simulink model "buck_ls_fault_sw_4rt"  (R2025a)
settings: Solver=VariableStepAuto  StartTime=0.0  StopTime=4  MaxStep=1/10e3  RelTol=1e-3
undefined symbols (not defined in the file or in its folder): plecs
settings Model: Creator=mem21  LastModifiedBy=mem21
settings DataIOCC: ReturnWorkspaceOutputs=off
settings OptimizationCC: DefaultParameterBehavior=Inlined  GainParamInheritBuiltInType=on  UseFloatMulNetSlope=on  InlineInvariantSignals=on  EfficientFloat2IntCast=on
settings DebuggingCC: SignalInfNanChecking=warning  AlgebraicLoopMsg=none
settings RTWCC: GenCodeOnly=on  BuildConfiguration=Faster Runs
settings GRTTargetCC: MatFileLogging=off  SupportNonFinite=off

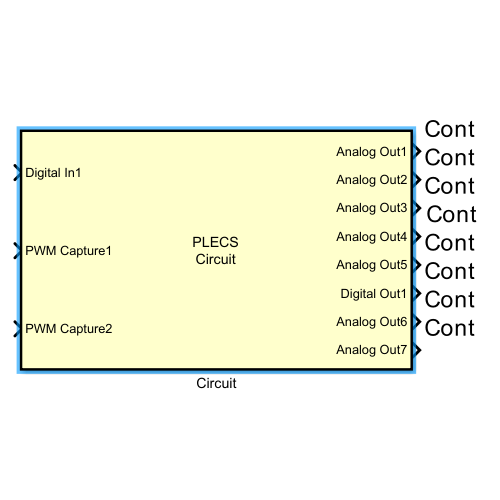
[thumbnail: Simulink's stored preview of the top-level diagram]
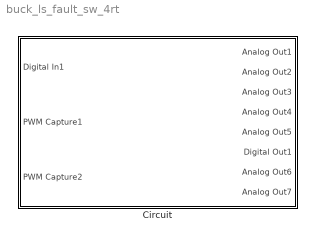
== system buck_ls_fault_sw_4rt ==
  Circuit : Subsystem  LoadFcn=plecs('sl', 200);  InitFcn=plecs('sl', 214);  StartFcn=plecs('sl', 208);  StopFcn=plecs('sl', 209);  mask(PlecsCircuit){PLECSData=<binary blob, 10120 chars, not shown>}
      mask prompts: PLECSData "PLECS Data (Do not delete or modify!)"
      mask init:
      | % PLACE CUSTOM INITIALIZATIONS ABOVE
      | % DO NOT REMOVE
      | plecs('sl', 215);
      | % DO NOT REMOVE
      settings: CopyFcn=plecs('sl', 203);  DeleteFcn=plecs('sl', 205);  UndoDeleteFcn=plecs('sl', 206);  PreSaveFcn=plecs('sl', 211);  PostSaveFcn=plecs('sl', 201);  NameChangeFcn=plecs('sl', 210);  DestroyFcn=plecs('sl', 207);  PreCopyFcn=plecs('sl', 216);  OpenFcn=plecs('sl', 202);  ErrorFcn=plerrorfcn
      mask Help: eval('plecs(''help'', ''qthelp:///creatingacircuit.html'')')
      mask Display: disp('PLECS\nCircuit')

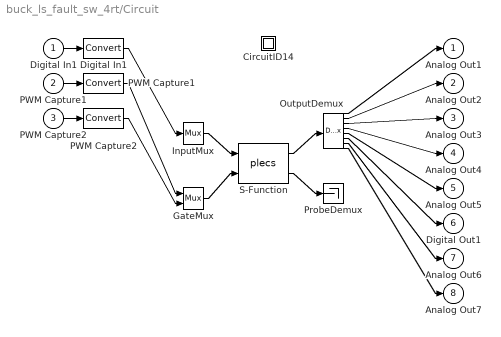
== system buck_ls_fault_sw_4rt/Circuit ==
  Digital In1 : Inport  PortDimensions=1
  PWM Capture1 : Inport  Port=2  PortDimensions=1
  PWM Capture2 : Inport  Port=3  PortDimensions=1
  " CircuitID14 " : Subsystem
  " Digital In1 " : DataTypeConversion
  " GateMux " : Mux  Inputs=[ 1 1 ]
  " InputMux " : Mux  Inputs=[ 1 ]
  " OutputDemux " : Demux  Outputs=[ 1 1 1 1 1 1 1 1 ]
  " PWM Capture1 " : DataTypeConversion
  " PWM Capture2 " : DataTypeConversion
  " ProbeDemux " : Terminator
  " S-Function " : S-Function  FunctionName=plecs  SFunctionDeploymentMode=off  EnableBusSupport=off
  Analog Out1 : Outport  PortDimensions=1
  Analog Out2 : Outport  Port=2  PortDimensions=1
  Analog Out3 : Outport  Port=3  PortDimensions=1
  Analog Out4 : Outport  Port=4  PortDimensions=1
  Analog Out5 : Outport  Port=5  PortDimensions=1
  Digital Out1 : Outport  Port=6  PortDimensions=1
  Analog Out6 : Outport  Port=7  PortDimensions=1
  Analog Out7 : Outport  Port=8  PortDimensions=1
  wires:
  " InputMux "/1 -> " S-Function "/1
  " GateMux "/1 -> " S-Function "/2
  " S-Function "/1 -> " OutputDemux "/1
  " S-Function "/2 -> " ProbeDemux "/1
  Digital In1/1 -> " Digital In1 "/1
  " Digital In1 "/1 -> " InputMux "/1
  PWM Capture1/1 -> " PWM Capture1 "/1
  " PWM Capture1 "/1 -> " GateMux "/1
  PWM Capture2/1 -> " PWM Capture2 "/1
  " PWM Capture2 "/1 -> " GateMux "/2
  " OutputDemux "/1 -> Analog Out1/1
  " OutputDemux "/2 -> Analog Out2/1
  " OutputDemux "/3 -> Analog Out3/1
  " OutputDemux "/4 -> Analog Out4/1
  " OutputDemux "/5 -> Analog Out5/1
  " OutputDemux "/6 -> Digital Out1/1
  " OutputDemux "/7 -> Analog Out6/1
  " OutputDemux "/8 -> Analog Out7/1

== system buck_ls_fault_sw_4rt/Circuit/ CircuitID14  ==
